simulink model "passband_72_channels_1"  (R2026a)
settings: Solver=VariableStepAuto  StopTime=0.3
libraries: commdigbbndpm3 x2, simulink x2, commfilt2 x2, commrandsrc3 x2, commchan3 x1, commsink2 x1, dspsigops x1
settings Model: Creator=MADHAV  LastModifiedBy=MADHAV

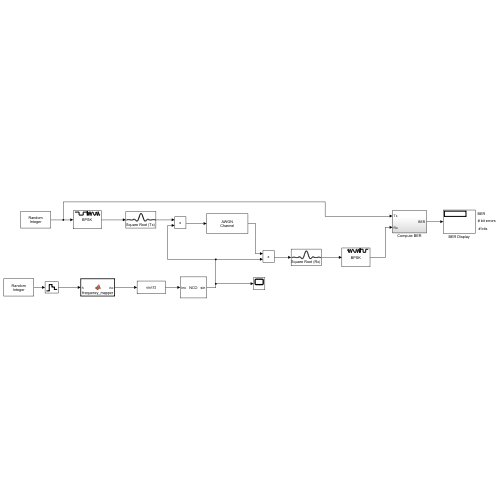
[thumbnail: Simulink's stored preview of the top-level diagram]
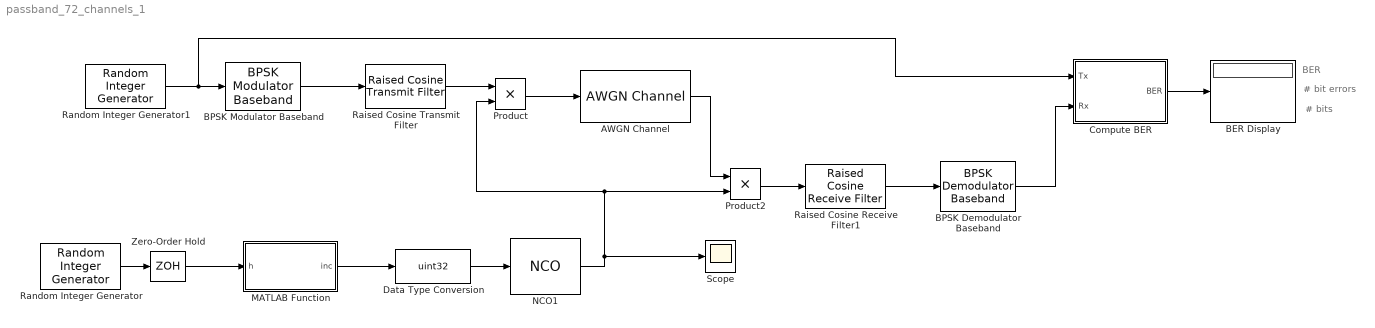
== system passband_72_channels_1 ==
  note: # bits
  note: BER
  note: # bit errors
  AWGN Channel : commchan3/AWGN Channel  LegacyMode=off  NoiseMethod="Signal to noise ratio  (SNR)"  noiseMode="Signal to noise ratio  (SNR)"  EbNo=10  EsNo=10  SNR=7  BitsPerSymbol=1  SignalPower=1  SpecifySymbolPeriod=off  SamplesPerSymbol=1  SymbolPeriod=1  VarianceSource=Parameter  Variance=1  RandomStream=Global stream  Seed=67  SimulateUsing=Code generation
  BER Display : Display
  BPSK Demodulator Baseband : commdigbbndpm3/BPSK Demodulator Baseband  DecType=Hard decision  VarSource=Dialog  Variance=1  Ph=0  outDtype=Inherit via internal rule  derotateFactorWordLen=16  derotateFactorDataTypeStr=Inherit: Same word length as input  derotateFactorLastDataTypeStr=Inherit: Same word length as input
      settings: LibrarySourceBlock=|
      | commhdldigbbndpm/BPSK
      | Demodulator
      | Baseband
  BPSK Modulator Baseband : commdigbbndpm3/BPSK Modulator Baseband  Ph=0  outDtype=double  outWordLen=16  outUDDataType=sfix(16)  outFracLenMode=Best precision  outFracLen=15  outDataTypeStr=double  outLastDataTypeStr=double
      settings: LibrarySourceBlock=|
      | commhdldigbbndpm/BPSK
      | Modulator
      | Baseband
  Compute BER : Subsystem
  Data Type Conversion : DataTypeConversion  OutDataTypeStr=uint32  SaturateOnIntegerOverflow=off  RndMeth=Floor
  MATLAB Function : MATLAB Function  TreatAsAtomicUnit=on
  NCO1 : dspsigops/NCO  AccIncSrc=Input port  AccInc=100  PhaseOffsetSrc=Specify via dialog  PhaseOffset=0  AccumWL=16  HasDither=on  DitherWL=4  PNgeneratorLength=19  HasPhaseQuantizer=on  TableDepth=12  HasOutputPhaseError=off  Formula=Sine  DataType=Binary point scaling  OutputWL=16  OutputFL=14  CompMethod=Table lookup (no interpolation)  SampleTime=1  SamplesPerFrame=1  OutputFrames=off
  Product : Product  RndMeth=Zero
  Product2 : Product
  Raised Cosine Receive Filter1 : commfilt2/Raised Cosine Receive Filter  filtType=Square root  R=0.2  filtSpan=8  N=8  downFactor=8  downOffset=0  filterGain=2  InputProcessing=Columns as channels (frame based)  RateOptions=Enforce single-rate processing  framing=Mute  checkCoeff=off  variableName=rcRxFilt1  currentFiltSpan=10  D=5  inputOffset=0  sampMode=Mute  saveAsFlag=0  rateMode=Downsampling  checkGain=Normalized  launchFVT=on  roundingMode=Floor  overflowMode=off  coeffDataTypeStr=Inherit: Same word length as input  coeffMin=[]  coeffMax=[]  coeffLastDataTypeStr=Inherit: Same word length as input  accumDataTypeStr=Inherit: Same as product output  accumLastDataTypeStr=Inherit: Same as product output  outputDataTypeStr=Inherit: Same as accumulator  outputMin=[]  outputMax=[]  outputLastDataTypeStr=Inherit: Same as accumulator
      settings: LibrarySourceBlock=|
      | commhdlfilt/Raised Cosine
      | Receive Filter
  Raised Cosine Transmit Filter : commfilt2/Raised Cosine Transmit Filter  filtType=Square root  R=0.2  filtSpan=8  N=8  filterGain=1  InputProcessing=Columns as channels (frame based)  RateOptions=Enforce single-rate processing  framing=Mute  checkCoeff=off  variableName=rcTxFilt1  checkGain=Normalized  sampMode=Mute  saveAsFlag=0  currentFiltSpan=2*(4)  D=4  launchFVT=off  roundingMode=Floor  overflowMode=off  coeffDataTypeStr=Inherit: Same word length as input  coeffMin=[]  coeffMax=[]  coeffLastDataTypeStr=Inherit: Same word length as input  outputDataTypeStr=Inherit: Same as accumulator  outputMin=[]  outputMax=[]  outputLastDataTypeStr=Inherit: Same as accumulator
  Random Integer Generator : commrandsrc3/Random Integer Generator  SetSize=71  SeedSource=Auto  Seed=12345  SampleTime=1e-3  SamplesPerFrame=1  OutputDataType=double  SimulateUsing=Interpreted execution
  Random Integer Generator1 : commrandsrc3/Random Integer Generator  SetSize=2  SeedSource=Parameter  Seed=37  SampleTime=1e-6  SamplesPerFrame=100  OutputDataType=double  SimulateUsing=Interpreted execution
  Scope : Scope
  Zero-Order Hold : ZeroOrderHold  SampleTime=5e-6
  wires:
  Zero-Order Hold/1 -> MATLAB Function/1(h)
  Data Type Conversion/1 -> NCO1/1
  Random Integer Generator/1 -> Zero-Order Hold/1
  MATLAB Function/1(inc) -> Data Type Conversion/1
  BPSK Demodulator Baseband/1 -> Compute BER/2(Rx)
  Raised Cosine Transmit Filter/1 -> Product/1
  Product2/1 -> Raised Cosine Receive Filter1/1
  AWGN Channel/1 -> Product2/1
  Compute BER/1(BER) -> BER Display/1
  BPSK Modulator Baseband/1 -> Raised Cosine Transmit Filter/1
  NCO1/1 -> Product/2, Product2/2, Scope/1
  Raised Cosine Receive Filter1/1 -> BPSK Demodulator Baseband/1
  Product/1 -> AWGN Channel/1
  Random Integer Generator1/1 -> Compute BER/1(Tx), BPSK Modulator Baseband/1

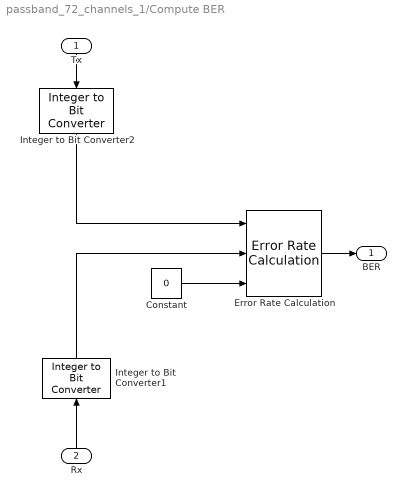
== system passband_72_channels_1/Compute BER ==
  Tx : Inport
  Rx : Inport  Port=2
  Constant : Constant  Value=0  SampleTime=1e-4
  Error Rate Calculation : commsink2/Error Rate Calculation  N=16  st_delay=0  cp_mode=Entire frame  subframe=[]  PMode=Port  WsName=ErrorVec  RsMode2=on  stop=off  numErr=100  maxBits=1e6
  Integer to Bit Converter1 : simulink/Logic and Bit Operations/Integer to Bit Converter  nbits=2  signedInputValues=Unsigned  bitOrder=MSB first  outDtype=boolean
  Integer to Bit Converter2 : simulink/Logic and Bit Operations/Integer to Bit Converter  nbits=2  signedInputValues=Unsigned  bitOrder=MSB first  outDtype=boolean
  BER : Outport  VectorParamsAs1DForOutWhenUnconnected=off
  wires:
  Integer to Bit Converter2/1 -> Error Rate Calculation/1
  Integer to Bit Converter1/1 -> Error Rate Calculation/2
  Tx/1 -> Integer to Bit Converter2/1
  Error Rate Calculation/1 -> BER/1
  Rx/1 -> Integer to Bit Converter1/1
  Constant/1 -> Error Rate Calculation/3

== matlab function passband_72_channels_1/MATLAB Function ==
  data: h input; inc output
function inc = frequency_mapper(h)

% Convert hop index (0 to 71) to frequency
f = 1000 + h*1000;

% Convert frequency to NCO phase increment
inc = floor(f*65536/200000);
